simulink model "Controller"  (R2018b)
settings: configuration reference "control_config" (kept outside this file)
values from neighbouring files (symbols this model uses):
  CONTROL_EXPORT = Simulink.Parameter(CONTROL_EXPORT_VALUE)    [controller_model_init.m]
  CONTROL_PARAM = Simulink.Parameter(CONTROL_PARAM_VALUE)    [controller_model_init.m]
undefined symbols (not defined in the file or in its folder): actuator_cmd, CONTROL_CONST, ControlMode, DiscIntNeverNeededParam, timestamp, VehicleStatus
libraries: simulink x27, FMT_Model_Lib x7
(part 2 of 3)

== system Controller/Controller/Control_Allocation/Quadcopter_x/Roll_Pitch_Remix ==
  Effective_Matrix : Inport
  torque_cmd : Inport  Port=2
  throttle_cmd : Inport  Port=3
  Constant : Constant  Value=up_lim  OutDataTypeStr=single
  Constant1 : Constant  Value=lo_lim  OutDataTypeStr=single
  Max : MinMax  Function=max
  Max1 : MinMax
  Multiply : Product  Multiplication=Matrix(*)  OutDataTypeStr=single
  Multiply1 : Product  OutDataTypeStr=single
  PQ_Remix : Subsystem
  Reshape : Reshape  OutputDimensionality=Column vector (2-D)
  Saturation3 : Saturate  UpperLimit=1  LowerLimit=0
  Saturation4 : Saturate  UpperLimit=1  LowerLimit=0
  Selector : Selector  InputPortWidth=3  IndexOptions=Index vector (dialog)  Indices=[1 2]  OutputSizes=1
  Sum : Sum  Inputs=|++
  Sum1 : Sum  Inputs=|++
  Sum2 : Sum  Inputs=|++
  pq_column : Selector  NumberOfDimensions=2  InputPortWidth=3  IndexOptions=Select all,Index vector (dialog)  Indices=[1:4],[1 2]  OutputSizes=1,1
  pq_remix_throttle : Outport
  wires:
  Multiply1/1 -> Sum2/1
  Multiply/1 -> Multiply1/1, Sum/1
  Constant1/1 -> PQ_Remix/4(lo_min)
  Sum/1 -> Max/1, Max1/1  "pq_premix"
  Max1/1 -> PQ_Remix/2(min)
  pq_column/1 -> Multiply/1
  Constant/1 -> PQ_Remix/3(up_lim)
  throttle_cmd/1 -> PQ_Remix/5(force_z_cmd), Sum/2, Sum1/2
  Reshape/1 -> Multiply/2
  Sum2/1 -> Saturation4/1  "pq_remix"
  Sum1/1 -> Saturation3/1
  PQ_Remix/1(roll_pitch_scale) -> Multiply1/2  "roll_pitch_scale"
  Saturation3/1 -> Sum2/2
  Selector/1 -> Reshape/1
  Saturation4/1 -> pq_remix_throttle/1
  Max/1 -> PQ_Remix/1(max)
  PQ_Remix/2(floating_throttle) -> Sum1/1  "floating_throttle"
  Effective_Matrix/1 -> pq_column/1
  torque_cmd/1 -> Selector/1

== system Controller/Controller/Control_Allocation/Quadcopter_x/Yaw_Remix ==
  Effective_Matrix : Inport
  torque_cmd : Inport  Port=2
  pq_remix : Inport  Port=3
  Constant : Constant  Value=up_lim  OutDataTypeStr=single
  Constant1 : Constant  Value=lo_lim  OutDataTypeStr=single
  Multiply2 : Product  Multiplication=Matrix(*)  OutDataTypeStr=single
  R_Remix : MATLAB Function  TreatAsAtomicUnit=on
  Selector2 : Selector  InputPortWidth=3  IndexOptions=Index vector (dialog)  Indices=3  OutputSizes=1
  Sum3 : Sum  Inputs=|++
  Sum4 : Sum  Inputs=++|
  r_column : Selector  NumberOfDimensions=2  InputPortWidth=3  IndexOptions=Select all,Index vector (dialog)  Indices=[1:4],3  OutputSizes=1,1
  pqr_remix_throttle : Outport
  wires:
  Sum4/1 -> pqr_remix_throttle/1  "pqr_remix"
  Selector2/1 -> Multiply2/2
  Effective_Matrix/1 -> r_column/1
  torque_cmd/1 -> Selector2/1
  r_column/1 -> R_Remix/3(r_column), Multiply2/1
  Sum3/1 -> Sum4/2, R_Remix/4(motor_out)
  Multiply2/1 -> Sum3/1
  pq_remix/1 -> Sum3/2
  Constant/1 -> R_Remix/1(up_lim)
  Constant1/1 -> R_Remix/2(lo_lim)
  R_Remix/1(floating_yaw) -> Sum4/1  "floating_yaw"

== system Controller/Controller/Control_Allocation/Quadcopter_x/actuator_cmd_routing ==
  throttle_cmd : Inport
  status : Inport  Port=2
  Constant : Constant  Value=zeros(12,1)  VectorParams1D=off  OutDataTypeStr=uint16
  Constant2 : Constant  Value=1000  OutDataTypeStr=uint32
  Data Type Conversion : DataTypeConversion  OutDataTypeStr=uint16
  Disarm : Constant  Value=ones(4,1)*1000  VectorParams1D=off  OutDataTypeStr=uint16
  Gain3 : Gain  Gain=1000  OutDataTypeStr=uint32
  Multiport Switch : MultiPortSwitch  DataPortForDefault=Additional data port  DiagnosticForDefault=None
  Mux1 : Mux  Inputs=2
  Reshape : Reshape  OutputDimensionality=Customize  OutputDimensions=[16,1]
  Saturation5 : Saturate  UpperLimit=1  LowerLimit=0
  Standby : Constant  Value=ones(4,1)*1150  VectorParams1D=off  OutDataTypeStr=uint16
  Sum5 : Sum  Inputs=|++
  actuator_cmd : Outport
  wires:
  Disarm/1 -> Multiport Switch/5, Multiport Switch/2
  Reshape/1 -> actuator_cmd/1
  Constant/1 -> Mux1/2
  Standby/1 -> Multiport Switch/3
  Mux1/1 -> Reshape/1
  status/1 -> Multiport Switch/1
  Multiport Switch/1 -> Mux1/1
  Sum5/1 -> Data Type Conversion/1
  Saturation5/1 -> Gain3/1
  Gain3/1 -> Sum5/1
  Constant2/1 -> Sum5/2
  throttle_cmd/1 -> Saturation5/1
  Data Type Conversion/1 -> Multiport Switch/4

== system Controller/Controller/Horizontal_Control/Attitude_Controller/Inner_Loop ==
  euler_rate_cmd_radPs : Inport
  INS_Out : Inport  Port=2
  FMS_Out : Inport  Port=3
  Bus Selector : BusSelector  OutputSignals=reset
  Rate_Controller : Subsystem
  Signal_Convert : Subsystem
  Signal_Select : Subsystem
  rate_dot_cmd_B : Outport
  wires:
  euler_rate_cmd_radPs/1 -> Signal_Convert/2(euler_rate_cmd)
  Signal_Select/1(out) -> Rate_Controller/1(rate_cmd_radPs)
  Rate_Controller/1(rate_dot_cmd_B) -> rate_dot_cmd_B/1
  Bus Selector/1 -> Rate_Controller/3(reset)  "<reset>"
  INS_Out/1 -> Signal_Convert/3(INS_Out), Rate_Controller/2(INS_Out)
  FMS_Out/1 -> Signal_Convert/1(FMS_Out), Bus Selector/1, Signal_Select/1(FMS_Out)
  Signal_Convert/1(rate_cmd_radPs) -> Signal_Select/2(rate_cmd_radPs)

== system Controller/Controller/Horizontal_Control/Attitude_Controller/Outter_Loop ==
  att_cmd_rad : Inport
  INS_Out : Inport  Port=2
  FMS_Out : Inport  Port=3
  Attitude_Controller : Subsystem
  Signal_Select : Subsystem
  euler_rate_cmd_radPs : Outport
  wires:
  Signal_Select/1(out) -> Attitude_Controller/1(att_cmd_rad)
  FMS_Out/1 -> Signal_Select/2(FMS_Out)
  INS_Out/1 -> Attitude_Controller/2(INS_Out)
  Attitude_Controller/1(euler_rate_cmd_radPs) -> euler_rate_cmd_radPs/1
  att_cmd_rad/1 -> Signal_Select/1(att_cmd_rad)

== system Controller/Controller/Horizontal_Control/Velocity_Controller/Accel_to_Attitude_CMD ==
  note: Gain to resist
      | air drag
  accel_cmd_C_mPs2 : Inport
  Atan : Trigonometry  Operator=atan
  Divide : Product  Inputs=*/
  Gain1 : Gain  Gain=-1
  Mux : Mux  Inputs=2
  Mux1 : Mux  Inputs=2
  Mux2 : Mux  Inputs=2
  Saturation : Saturate  UpperLimit=CONTROL_PARAM.MC_ROLL_PITCH_LIM  LowerLimit=-CONTROL_PARAM.MC_ROLL_PITCH_LIM
  Selector : Selector  InputPortWidth=2  IndexOptions=Index vector (dialog)  Indices=1  OutputSizes=1
  Selector1 : Selector  InputPortWidth=2  IndexOptions=Index vector (dialog)  Indices=2  OutputSizes=1
  Vector Modulus : FMT_Model_Lib/Math/Vector Modulus
      settings: SourceProductName=FMT Toolbox
  g : Constant  Value=9.8055  OutDataTypeStr=single
  gain : Gain  Gain=1.1
  att_cmd_B_rad : Outport
  wires:
  Atan/1 -> Saturation/1
  g/1 -> Mux2/2, Mux1/1
  Divide/1 -> Atan/1
  Selector/1 -> Gain1/1
  gain/1 -> Selector1/1, Selector/1
  Gain1/1 -> Mux/2
  Saturation/1 -> att_cmd_B_rad/1
  Mux1/1 -> Divide/2
  Vector Modulus/1 -> Mux1/2
  Selector1/1 -> Mux2/1, Mux/1
  accel_cmd_C_mPs2/1 -> gain/1
  Mux/1 -> Divide/1
  Mux2/1 -> Vector Modulus/1

== system Controller/Controller/Horizontal_Control/Velocity_Controller/Error ==
  INS_Out : Inport
  FMS_Out : Inport  Port=2
  Bus Selector : BusSelector  OutputSignals=u_cmd,v_cmd
  Bus Selector1 : BusSelector  OutputSignals=flag
  Bus_Select : Subsystem
  Compare To Zero : simulink/Logic and Bit Operations/Compare To Zero  relop===  OutDataTypeStr=boolean
  Mux : Mux  Inputs=2
  Sum : Sum  Inputs=|+-
  Switch : Switch  Criteria=u2 > Threshold
  TD : Subsystem
  vel_valid : simulink/Logic and Bit Operations/Bitwise Operator  logicop=AND  UseBitMask=on  BitMask=bin2dec('10000')  BitMaskRealWorld=Stored Integer
  uv_err_C_mPs : Outport
  wires:
  FMS_Out/1 -> Bus Selector/1
  INS_Out/1 -> Bus Selector1/1, Bus_Select/1(INS_Out)
  Bus Selector/1 -> Mux/1  "<u_cmd>"
  Bus Selector/2 -> Mux/2  "<v_cmd>"
  Mux/1 -> Switch/1, TD/1(v)  "uv_cmd_C_mPs"
  Bus_Select/1(uv_est_C_mPs) -> Switch/3, Sum/2  "uv_est_C_mPs"
  Sum/1 -> uv_err_C_mPs/1  "uv_error_C_mPs"
  Bus Selector1/1 -> vel_valid/1  "<flag>"
  Switch/1 -> TD/2(v0)
  vel_valid/1 -> Compare To Zero/1
  Compare To Zero/1 -> Switch/2
  TD/1(v1) -> Sum/1  "uv_cmd_C_mPs"

== system Controller/Controller/Horizontal_Control/Velocity_Controller/PID_Controller ==
  uv_err_C_mPs : Inport
  reset : Inport  Port=2
  Add : Sum  Inputs=+++
  D_Control : Subsystem  mask{kd=CONTROL_PARAM.MC_VEL_XY_D, max_d=CONTROL_PARAM.MC_VEL_XY_D_MAX, min_d=CONTROL_PARAM.MC_VEL_XY_D_MIN}
  I_Control : Subsystem  mask{ki=CONTROL_PARAM.MC_VEL_XY_I, max_i=CONTROL_PARAM.MC_VEL_XY_I_MAX, min_i=CONTROL_PARAM.MC_VEL_XY_I_MIN}
  P_Control : Subsystem  mask{kp=CONTROL_PARAM.MC_VEL_XY_P}
  accel_cmd_C : Outport
  wires:
  uv_err_C_mPs/1 -> P_Control/1(err), I_Control/1(err), D_Control/1(err)
  reset/1 -> I_Control/2(reset), D_Control/2(reset)
  P_Control/1(p_out) -> Add/1  "accel_p_out"
  I_Control/1(i_out) -> Add/2  "accel_i_out"
  D_Control/1(d_out) -> Add/3  "accel_d_out"
  Add/1 -> accel_cmd_C/1

== system Controller/Controller/Horizontal_Control/Velocity_Controller/Signal_Select ==
  acc_cmd_in : Inport
  FMS_Out : Inport  Port=2
  Bus Selector : BusSelector  OutputSignals=ctrl_mode
  Offboard : simulink/Logic and Bit Operations/Compare To Constant  relop===  const=uint8(ControlMode.Offboard)  OutDataTypeStr=boolean
  Offboard_Signal_Select : Subsystem
  Switch : Switch  Criteria=u2 > Threshold
  acc_cmd_out : Outport
  wires:
  FMS_Out/1 -> Offboard_Signal_Select/1(FMS_Out), Bus Selector/1
  Bus Selector/1 -> Offboard/1  "<ctrl_mode>"
  Offboard/1 -> Switch/2
  Switch/1 -> acc_cmd_out/1
  acc_cmd_in/1 -> Offboard_Signal_Select/2(acc_cmd_in), Switch/3
  Offboard_Signal_Select/1(acc_cmd) -> Switch/1

== system Controller/Controller/Vertical_Control/Signal_Select/Offboard_Signal_Select ==
  FMS_Out : Inport
  throttle_cmd_in : Inport  Port=2
  Bias : Bias  Bias=-1
  Bus Selector1 : BusSelector  OutputSignals=cmd_mask
  Bus Selector2 : BusSelector  OutputSignals=throttle_cmd
  Gain : Gain  Gain=1/1000  OutDataTypeStr=single
  Switch : Switch  Criteria=u2 > Threshold
  cmd_throttle valid : simulink/Logic and Bit Operations/Bitwise Operator  logicop=AND  UseBitMask=on  BitMask=bin2dec('1000000000000')  BitMaskRealWorld=Stored Integer
  throttle_cmd_out : Outport
  wires:
  Switch/1 -> throttle_cmd_out/1
  cmd_throttle valid/1 -> Switch/2
  FMS_Out/1 -> Bus Selector2/1, Bus Selector1/1
  Bus Selector1/1 -> cmd_throttle valid/1  "<cmd_mask>"
  Bus Selector2/1 -> Gain/1  "<throttle_cmd>"
  throttle_cmd_in/1 -> Switch/3
  Gain/1 -> Bias/1
  Bias/1 -> Switch/1

== system Controller/Controller/Vertical_Control/Veloxity_Z_Controller/Boosted_Throttle ==
  thrust_cmd : Inport
  INS_Out : Inport  Port=2
  Bus Selector : BusSelector  OutputSignals=phi,theta
  Constant : Constant  OutDataTypeStr=single
  Cos : Trigonometry  Operator=cos
  Cos1 : Trigonometry  Operator=cos
  Divide : Product  Inputs=*/
  Gain : Gain  Gain=2
  Multiply : Product
  Multiply1 : Product  Inputs=3
  Saturation : Saturate  UpperLimit=1  LowerLimit=0
  Saturation1 : Saturate  UpperLimit=1  LowerLimit=0.5
  boosted_thrust : Outport
  wires:
  INS_Out/1 -> Bus Selector/1
  Bus Selector/1 -> Cos/1  "<phi>"
  Bus Selector/2 -> Cos1/1  "<theta>"
  Cos/1 -> Multiply/1
  Cos1/1 -> Multiply/2
  Multiply/1 -> Saturation1/1, Gain/1
  Gain/1 -> Saturation/1
  Saturation/1 -> Multiply1/3  "inverted_factor"
  Constant/1 -> Divide/1
  Divide/1 -> Multiply1/2  "boost_factor"
  Saturation1/1 -> Divide/2
  thrust_cmd/1 -> Multiply1/1
  Multiply1/1 -> boosted_thrust/1

== system Controller/Controller/Vertical_Control/Veloxity_Z_Controller/Error ==
  FMS_Out : Inport
  INS_Out : Inport  Port=2
  Bus Selector1 : BusSelector  OutputSignals=vd
  Bus Selector2 : BusSelector  OutputSignals=w_cmd
  Bus Selector3 : BusSelector  OutputSignals=flag
  Compare To Zero : simulink/Logic and Bit Operations/Compare To Zero  relop===  OutDataTypeStr=boolean
  Gain : Gain  Gain=-1  OutDataTypeStr=Inherit: Same as input
  Signal Copy1 : SignalConversion  OverrideOpt=off
  Sum1 : Sum  Inputs=|+-
  Switch : Switch  Criteria=u2 > Threshold
  TD : Subsystem
  vel_valid : simulink/Logic and Bit Operations/Bitwise Operator  logicop=AND  UseBitMask=on  BitMask=bin2dec('10000')  BitMaskRealWorld=Stored Integer
  az_cmd_C_mPs2 : Outport
  wires:
  Sum1/1 -> Gain/1  "w_error_C_mPs"
  FMS_Out/1 -> Bus Selector2/1
  TD/1(v1) -> Sum1/1  "w_cmd_C_mPs"
  Signal Copy1/1 -> Sum1/2  "w_est_C_mPs"
  Bus Selector2/1 -> Switch/1, TD/1(v)  "<w_cmd>"
  Gain/1 -> az_cmd_C_mPs2/1
  vel_valid/1 -> Compare To Zero/1
  Compare To Zero/1 -> Switch/2
  INS_Out/1 -> Bus Selector3/1, Bus Selector1/1
  Bus Selector3/1 -> vel_valid/1  "<flag>"
  Bus Selector1/1 -> Switch/3, Signal Copy1/1  "<vd>"
  Switch/1 -> TD/2(v0)

== system Controller/Controller/Vertical_Control/Veloxity_Z_Controller/PID_Controller ==
  az_cmd_C_mPs2 : Inport
  reset : Inport  Port=2
  prev_status : Inport  Port=3
  Add : Sum  Inputs=+++
  Compare To Constant : simulink/Logic and Bit Operations/Compare To Constant  relop=<  const=uint8(VehicleStatus.Arm)  OutDataTypeStr=boolean
  D_Control : Subsystem  mask{kd=CONTROL_PARAM.MC_VEL_Z_D, max_d=CONTROL_PARAM.MC_VEL_Z_D_MAX, min_d=CONTROL_PARAM.MC_VEL_Z_D_MIN}
  I_Control : Subsystem  mask{ki=CONTROL_PARAM.MC_VEL_Z_I, max_i=CONTROL_PARAM.MC_VEL_Z_I_MAX, min_i=CONTROL_PARAM.MC_VEL_Z_I_MIN}
  P_Control : Subsystem  mask{kp=CONTROL_PARAM.MC_VEL_Z_P}
  thrust_cmd : Outport
  wires:
  P_Control/1(p_out) -> Add/1  "thrust_p_out"
  I_Control/1(i_out) -> Add/2  "thrust_i_out"
  Add/1 -> thrust_cmd/1
  az_cmd_C_mPs2/1 -> D_Control/1(err), I_Control/1(err), P_Control/1(err)
  D_Control/1(d_out) -> Add/3  "thrust_d_out"
  Compare To Constant/1 -> I_Control/2(slow_start)
  reset/1 -> D_Control/2(reset), I_Control/3(reset)
  prev_status/1 -> Compare To Constant/1

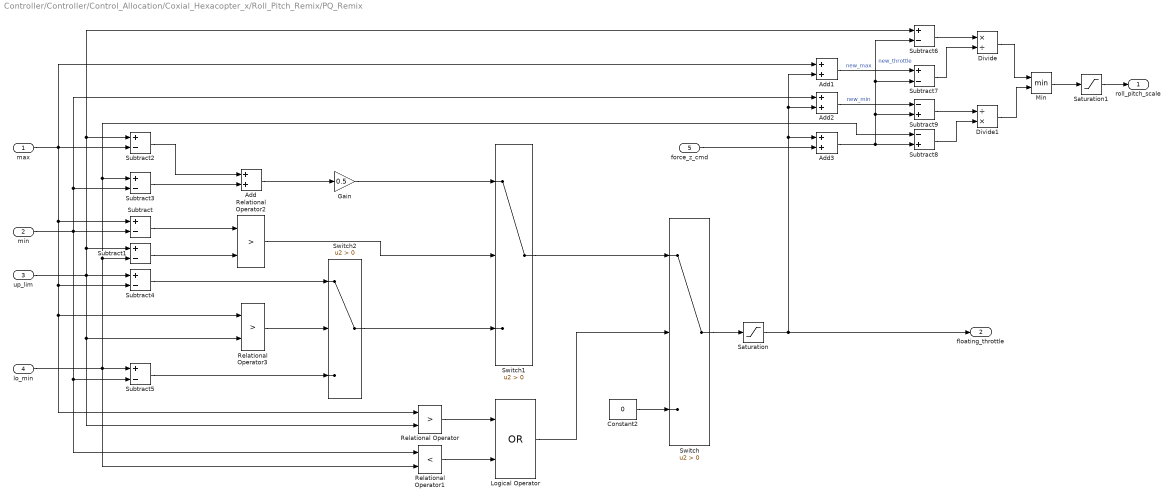
== system Controller/Controller/Control_Allocation/Coxial_Hexacopter_x/Roll_Pitch_Remix/PQ_Remix ==
  max : Inport
  min : Inport  Port=2
  up_lim : Inport  Port=3
  lo_min : Inport  Port=4
  force_z_cmd : Inport  Port=5
  Add{,1..3} (4 alike) : Sum
  Constant2 : Constant  Value=0  OutDataTypeStr=single
  Divide : Product  Inputs=*/
  Divide1 : Product  Inputs=/*
  Gain : Gain  Gain=0.5
  Logical Operator : Logic  Operator=OR  AllPortsSameDT=off  OutDataTypeStr=boolean
  Min : MinMax  Inputs=2
  Relational Operator : RelationalOperator  Operator=>  OutDataTypeStr=boolean  RndMeth=Simplest
  Relational Operator1 : RelationalOperator  Operator=<  OutDataTypeStr=boolean  RndMeth=Simplest
  Relational Operator2 : RelationalOperator  Operator=>  OutDataTypeStr=boolean  RndMeth=Simplest
  Relational Operator3 : RelationalOperator  Operator=>  OutDataTypeStr=boolean  RndMeth=Simplest
  Saturation : Saturate  UpperLimit=0.2  LowerLimit=-0.2
  Saturation1 : Saturate  UpperLimit=1  LowerLimit=0.5
  Subtract{,1..7} (8 alike) : Sum  Inputs=+-
  Subtract8 : Sum  Inputs=-+
  Subtract9 : Sum  Inputs=-+
  Switch : Switch  Criteria=u2 > Threshold
  Switch1 : Switch  Criteria=u2 > Threshold
  Switch2 : Switch  Criteria=u2 > Threshold
  roll_pitch_scale : Outport
  floating_throttle : Outport  Port=2
  wires:
  max/1 -> Subtract/1, Relational Operator3/1, Relational Operator/1, Subtract4/2, Add1/1, Subtract2/2
  up_lim/1 -> Relational Operator/2, Relational Operator3/2, Subtract6/1, Subtract2/1, Subtract1/1, Subtract4/1
  min/1 -> Add2/1, Subtract3/2, Subtract/2, Relational Operator1/1, Subtract5/2
  lo_min/1 -> Subtract8/1, Subtract3/1, Subtract1/2, Relational Operator1/2, Subtract5/1
  Relational Operator/1 -> Logical Operator/1
  Relational Operator1/1 -> Logical Operator/2
  Logical Operator/1 -> Switch/2
  Constant2/1 -> Switch/3
  Subtract/1 -> Relational Operator2/1
  Subtract1/1 -> Relational Operator2/2
  Relational Operator2/1 -> Switch1/2
  Subtract2/1 -> Add/1
  Subtract3/1 -> Add/2
  Add/1 -> Gain/1
  Gain/1 -> Switch1/1
  Relational Operator3/1 -> Switch2/2
  Subtract4/1 -> Switch2/1
  Switch1/1 -> Switch/1
  Switch2/1 -> Switch1/3
  Subtract5/1 -> Switch2/3
  Switch/1 -> Saturation/1
  force_z_cmd/1 -> Add3/2
  Add1/1 -> Subtract7/1  "new_max"
  Add2/1 -> Subtract9/1  "new_min"
  Add3/1 -> Subtract7/2, Subtract6/2, Subtract9/2, Subtract8/2  "new_throttle"
  Subtract6/1 -> Divide/1
  Subtract7/1 -> Divide/2
  Subtract8/1 -> Divide1/2
  Subtract9/1 -> Divide1/1
  Divide/1 -> Min/1
  Divide1/1 -> Min/2
  Min/1 -> Saturation1/1
  Saturation1/1 -> roll_pitch_scale/1
  Saturation/1 -> Add3/1, Add2/2, Add1/2, floating_throttle/1

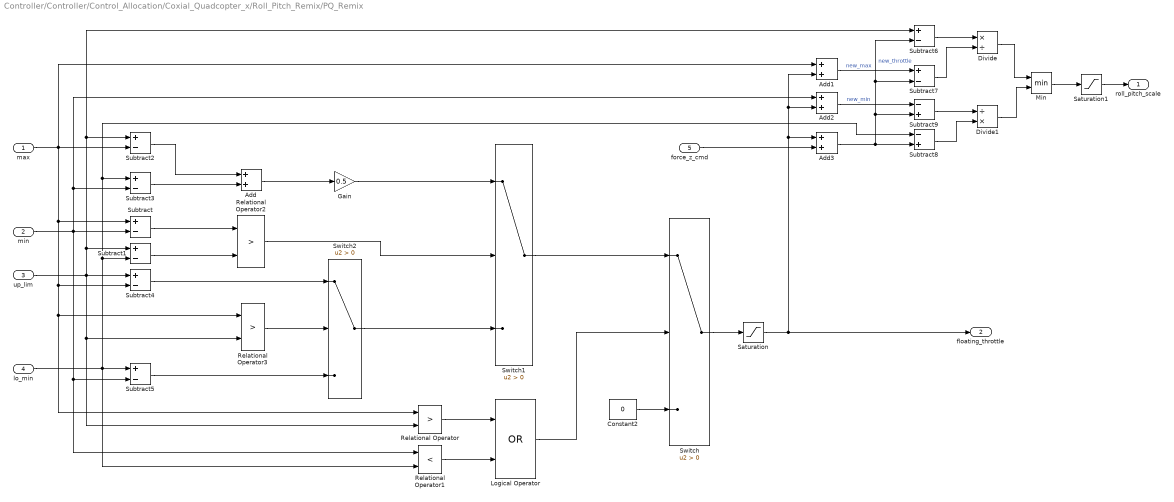
== system Controller/Controller/Control_Allocation/Coxial_Quadcopter_x/Roll_Pitch_Remix/PQ_Remix ==
  max : Inport
  min : Inport  Port=2
  up_lim : Inport  Port=3
  lo_min : Inport  Port=4
  force_z_cmd : Inport  Port=5
  Add{,1..3} (4 alike) : Sum
  Constant2 : Constant  Value=0  OutDataTypeStr=single
  Divide : Product  Inputs=*/
  Divide1 : Product  Inputs=/*
  Gain : Gain  Gain=0.5
  Logical Operator : Logic  Operator=OR  AllPortsSameDT=off  OutDataTypeStr=boolean
  Min : MinMax  Inputs=2
  Relational Operator : RelationalOperator  Operator=>  OutDataTypeStr=boolean  RndMeth=Simplest
  Relational Operator1 : RelationalOperator  Operator=<  OutDataTypeStr=boolean  RndMeth=Simplest
  Relational Operator2 : RelationalOperator  Operator=>  OutDataTypeStr=boolean  RndMeth=Simplest
  Relational Operator3 : RelationalOperator  Operator=>  OutDataTypeStr=boolean  RndMeth=Simplest
  Saturation : Saturate  UpperLimit=0.2  LowerLimit=-0.2
  Saturation1 : Saturate  UpperLimit=1  LowerLimit=0.5
  Subtract{,1..7} (8 alike) : Sum  Inputs=+-
  Subtract8 : Sum  Inputs=-+
  Subtract9 : Sum  Inputs=-+
  Switch : Switch  Criteria=u2 > Threshold
  Switch1 : Switch  Criteria=u2 > Threshold
  Switch2 : Switch  Criteria=u2 > Threshold
  roll_pitch_scale : Outport
  floating_throttle : Outport  Port=2
  wires:
  max/1 -> Subtract/1, Relational Operator3/1, Relational Operator/1, Subtract4/2, Add1/1, Subtract2/2
  up_lim/1 -> Relational Operator/2, Relational Operator3/2, Subtract6/1, Subtract2/1, Subtract1/1, Subtract4/1
  min/1 -> Add2/1, Subtract3/2, Subtract/2, Relational Operator1/1, Subtract5/2
  lo_min/1 -> Subtract8/1, Subtract3/1, Subtract1/2, Relational Operator1/2, Subtract5/1
  Relational Operator/1 -> Logical Operator/1
  Relational Operator1/1 -> Logical Operator/2
  Logical Operator/1 -> Switch/2
  Constant2/1 -> Switch/3
  Subtract/1 -> Relational Operator2/1
  Subtract1/1 -> Relational Operator2/2
  Relational Operator2/1 -> Switch1/2
  Subtract2/1 -> Add/1
  Subtract3/1 -> Add/2
  Add/1 -> Gain/1
  Gain/1 -> Switch1/1
  Relational Operator3/1 -> Switch2/2
  Subtract4/1 -> Switch2/1
  Switch1/1 -> Switch/1
  Switch2/1 -> Switch1/3
  Subtract5/1 -> Switch2/3
  Switch/1 -> Saturation/1
  force_z_cmd/1 -> Add3/2
  Add1/1 -> Subtract7/1  "new_max"
  Add2/1 -> Subtract9/1  "new_min"
  Add3/1 -> Subtract7/2, Subtract6/2, Subtract9/2, Subtract8/2  "new_throttle"
  Subtract6/1 -> Divide/1
  Subtract7/1 -> Divide/2
  Subtract8/1 -> Divide1/2
  Subtract9/1 -> Divide1/1
  Divide/1 -> Min/1
  Divide1/1 -> Min/2
  Min/1 -> Saturation1/1
  Saturation1/1 -> roll_pitch_scale/1
  Saturation/1 -> Add3/1, Add2/2, Add1/2, floating_throttle/1

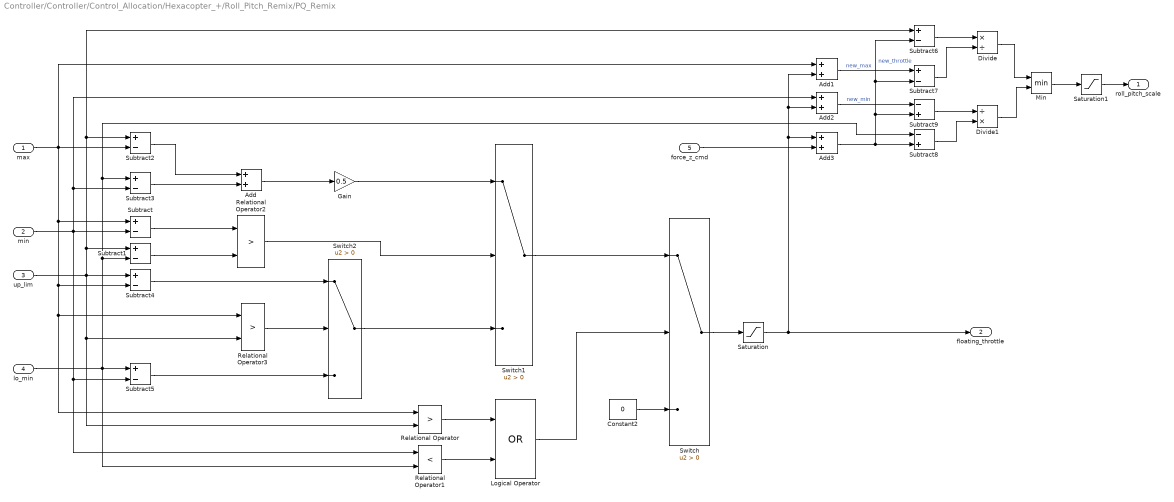
== system Controller/Controller/Control_Allocation/Hexacopter_+/Roll_Pitch_Remix/PQ_Remix ==
  max : Inport
  min : Inport  Port=2
  up_lim : Inport  Port=3
  lo_min : Inport  Port=4
  force_z_cmd : Inport  Port=5
  Add{,1..3} (4 alike) : Sum
  Constant2 : Constant  Value=0  OutDataTypeStr=single
  Divide : Product  Inputs=*/
  Divide1 : Product  Inputs=/*
  Gain : Gain  Gain=0.5
  Logical Operator : Logic  Operator=OR  AllPortsSameDT=off  OutDataTypeStr=boolean
  Min : MinMax  Inputs=2
  Relational Operator : RelationalOperator  Operator=>  OutDataTypeStr=boolean  RndMeth=Simplest
  Relational Operator1 : RelationalOperator  Operator=<  OutDataTypeStr=boolean  RndMeth=Simplest
  Relational Operator2 : RelationalOperator  Operator=>  OutDataTypeStr=boolean  RndMeth=Simplest
  Relational Operator3 : RelationalOperator  Operator=>  OutDataTypeStr=boolean  RndMeth=Simplest
  Saturation : Saturate  UpperLimit=0.2  LowerLimit=-0.2
  Saturation1 : Saturate  UpperLimit=1  LowerLimit=0.5
  Subtract{,1..7} (8 alike) : Sum  Inputs=+-
  Subtract8 : Sum  Inputs=-+
  Subtract9 : Sum  Inputs=-+
  Switch : Switch  Criteria=u2 > Threshold
  Switch1 : Switch  Criteria=u2 > Threshold
  Switch2 : Switch  Criteria=u2 > Threshold
  roll_pitch_scale : Outport
  floating_throttle : Outport  Port=2
  wires:
  max/1 -> Subtract/1, Relational Operator3/1, Relational Operator/1, Subtract4/2, Add1/1, Subtract2/2
  up_lim/1 -> Relational Operator/2, Relational Operator3/2, Subtract6/1, Subtract2/1, Subtract1/1, Subtract4/1
  min/1 -> Add2/1, Subtract3/2, Subtract/2, Relational Operator1/1, Subtract5/2
  lo_min/1 -> Subtract8/1, Subtract3/1, Subtract1/2, Relational Operator1/2, Subtract5/1
  Relational Operator/1 -> Logical Operator/1
  Relational Operator1/1 -> Logical Operator/2
  Logical Operator/1 -> Switch/2
  Constant2/1 -> Switch/3
  Subtract/1 -> Relational Operator2/1
  Subtract1/1 -> Relational Operator2/2
  Relational Operator2/1 -> Switch1/2
  Subtract2/1 -> Add/1
  Subtract3/1 -> Add/2
  Add/1 -> Gain/1
  Gain/1 -> Switch1/1
  Relational Operator3/1 -> Switch2/2
  Subtract4/1 -> Switch2/1
  Switch1/1 -> Switch/1
  Switch2/1 -> Switch1/3
  Subtract5/1 -> Switch2/3
  Switch/1 -> Saturation/1
  force_z_cmd/1 -> Add3/2
  Add1/1 -> Subtract7/1  "new_max"
  Add2/1 -> Subtract9/1  "new_min"
  Add3/1 -> Subtract7/2, Subtract6/2, Subtract9/2, Subtract8/2  "new_throttle"
  Subtract6/1 -> Divide/1
  Subtract7/1 -> Divide/2
  Subtract8/1 -> Divide1/2
  Subtract9/1 -> Divide1/1
  Divide/1 -> Min/1
  Divide1/1 -> Min/2
  Min/1 -> Saturation1/1
  Saturation1/1 -> roll_pitch_scale/1
  Saturation/1 -> Add3/1, Add2/2, Add1/2, floating_throttle/1

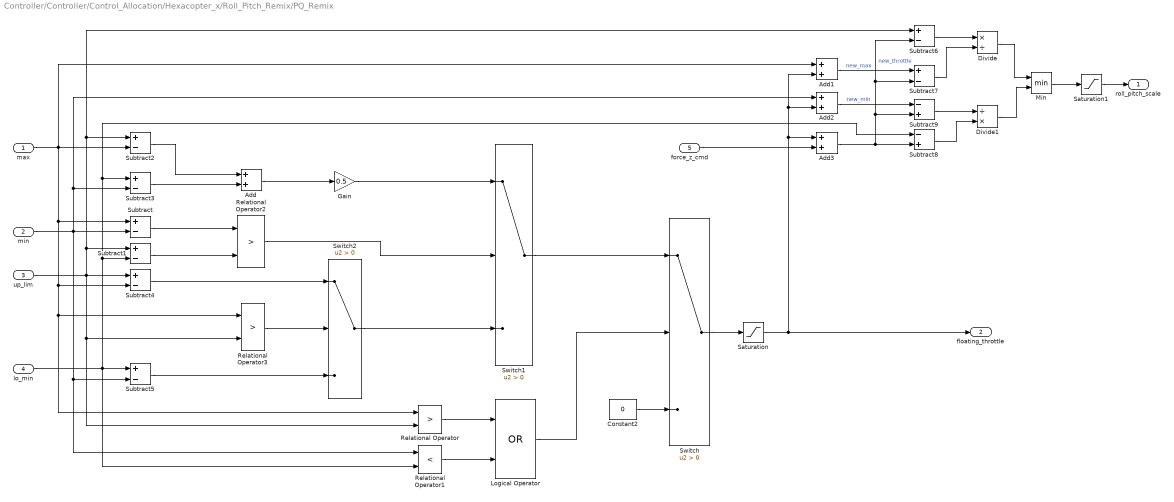
== system Controller/Controller/Control_Allocation/Hexacopter_x/Roll_Pitch_Remix/PQ_Remix ==
  max : Inport
  min : Inport  Port=2
  up_lim : Inport  Port=3
  lo_min : Inport  Port=4
  force_z_cmd : Inport  Port=5
  Add{,1..3} (4 alike) : Sum
  Constant2 : Constant  Value=0  OutDataTypeStr=single
  Divide : Product  Inputs=*/
  Divide1 : Product  Inputs=/*
  Gain : Gain  Gain=0.5
  Logical Operator : Logic  Operator=OR  AllPortsSameDT=off  OutDataTypeStr=boolean
  Min : MinMax  Inputs=2
  Relational Operator : RelationalOperator  Operator=>  OutDataTypeStr=boolean  RndMeth=Simplest
  Relational Operator1 : RelationalOperator  Operator=<  OutDataTypeStr=boolean  RndMeth=Simplest
  Relational Operator2 : RelationalOperator  Operator=>  OutDataTypeStr=boolean  RndMeth=Simplest
  Relational Operator3 : RelationalOperator  Operator=>  OutDataTypeStr=boolean  RndMeth=Simplest
  Saturation : Saturate  UpperLimit=0.2  LowerLimit=-0.2
  Saturation1 : Saturate  UpperLimit=1  LowerLimit=0.5
  Subtract{,1..7} (8 alike) : Sum  Inputs=+-
  Subtract8 : Sum  Inputs=-+
  Subtract9 : Sum  Inputs=-+
  Switch : Switch  Criteria=u2 > Threshold
  Switch1 : Switch  Criteria=u2 > Threshold
  Switch2 : Switch  Criteria=u2 > Threshold
  roll_pitch_scale : Outport
  floating_throttle : Outport  Port=2
  wires:
  max/1 -> Subtract/1, Relational Operator3/1, Relational Operator/1, Subtract4/2, Add1/1, Subtract2/2
  up_lim/1 -> Relational Operator/2, Relational Operator3/2, Subtract6/1, Subtract2/1, Subtract1/1, Subtract4/1
  min/1 -> Add2/1, Subtract3/2, Subtract/2, Relational Operator1/1, Subtract5/2
  lo_min/1 -> Subtract8/1, Subtract3/1, Subtract1/2, Relational Operator1/2, Subtract5/1
  Relational Operator/1 -> Logical Operator/1
  Relational Operator1/1 -> Logical Operator/2
  Logical Operator/1 -> Switch/2
  Constant2/1 -> Switch/3
  Subtract/1 -> Relational Operator2/1
  Subtract1/1 -> Relational Operator2/2
  Relational Operator2/1 -> Switch1/2
  Subtract2/1 -> Add/1
  Subtract3/1 -> Add/2
  Add/1 -> Gain/1
  Gain/1 -> Switch1/1
  Relational Operator3/1 -> Switch2/2
  Subtract4/1 -> Switch2/1
  Switch1/1 -> Switch/1
  Switch2/1 -> Switch1/3
  Subtract5/1 -> Switch2/3
  Switch/1 -> Saturation/1
  force_z_cmd/1 -> Add3/2
  Add1/1 -> Subtract7/1  "new_max"
  Add2/1 -> Subtract9/1  "new_min"
  Add3/1 -> Subtract7/2, Subtract6/2, Subtract9/2, Subtract8/2  "new_throttle"
  Subtract6/1 -> Divide/1
  Subtract7/1 -> Divide/2
  Subtract8/1 -> Divide1/2
  Subtract9/1 -> Divide1/1
  Divide/1 -> Min/1
  Divide1/1 -> Min/2
  Min/1 -> Saturation1/1
  Saturation1/1 -> roll_pitch_scale/1
  Saturation/1 -> Add3/1, Add2/2, Add1/2, floating_throttle/1

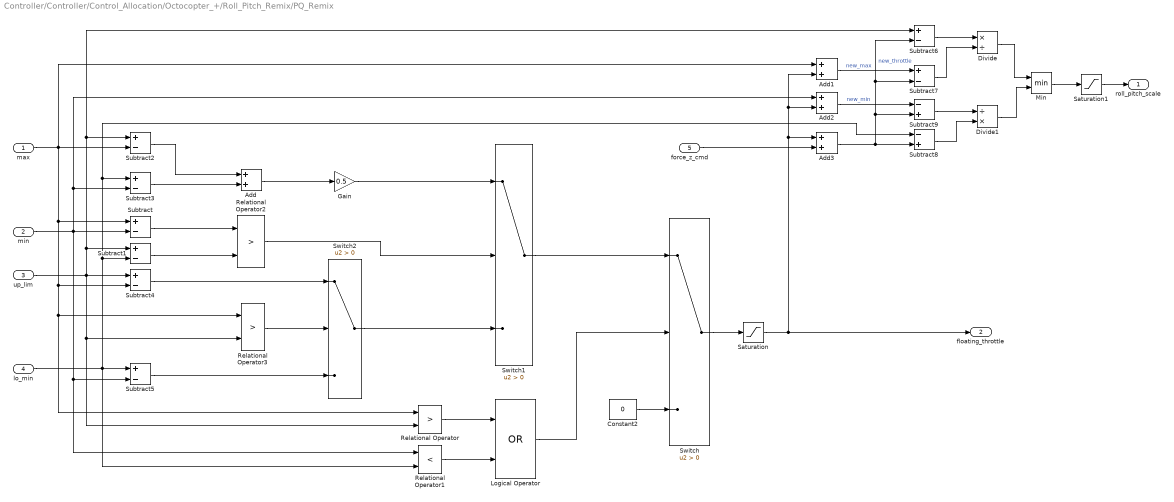
== system Controller/Controller/Control_Allocation/Octocopter_+/Roll_Pitch_Remix/PQ_Remix ==
  max : Inport
  min : Inport  Port=2
  up_lim : Inport  Port=3
  lo_min : Inport  Port=4
  force_z_cmd : Inport  Port=5
  Add{,1..3} (4 alike) : Sum
  Constant2 : Constant  Value=0  OutDataTypeStr=single
  Divide : Product  Inputs=*/
  Divide1 : Product  Inputs=/*
  Gain : Gain  Gain=0.5
  Logical Operator : Logic  Operator=OR  AllPortsSameDT=off  OutDataTypeStr=boolean
  Min : MinMax  Inputs=2
  Relational Operator : RelationalOperator  Operator=>  OutDataTypeStr=boolean  RndMeth=Simplest
  Relational Operator1 : RelationalOperator  Operator=<  OutDataTypeStr=boolean  RndMeth=Simplest
  Relational Operator2 : RelationalOperator  Operator=>  OutDataTypeStr=boolean  RndMeth=Simplest
  Relational Operator3 : RelationalOperator  Operator=>  OutDataTypeStr=boolean  RndMeth=Simplest
  Saturation : Saturate  UpperLimit=0.2  LowerLimit=-0.2
  Saturation1 : Saturate  UpperLimit=1  LowerLimit=0.5
  Subtract{,1..7} (8 alike) : Sum  Inputs=+-
  Subtract8 : Sum  Inputs=-+
  Subtract9 : Sum  Inputs=-+
  Switch : Switch  Criteria=u2 > Threshold
  Switch1 : Switch  Criteria=u2 > Threshold
  Switch2 : Switch  Criteria=u2 > Threshold
  roll_pitch_scale : Outport
  floating_throttle : Outport  Port=2
  wires:
  max/1 -> Subtract/1, Relational Operator3/1, Relational Operator/1, Subtract4/2, Add1/1, Subtract2/2
  up_lim/1 -> Relational Operator/2, Relational Operator3/2, Subtract6/1, Subtract2/1, Subtract1/1, Subtract4/1
  min/1 -> Add2/1, Subtract3/2, Subtract/2, Relational Operator1/1, Subtract5/2
  lo_min/1 -> Subtract8/1, Subtract3/1, Subtract1/2, Relational Operator1/2, Subtract5/1
  Relational Operator/1 -> Logical Operator/1
  Relational Operator1/1 -> Logical Operator/2
  Logical Operator/1 -> Switch/2
  Constant2/1 -> Switch/3
  Subtract/1 -> Relational Operator2/1
  Subtract1/1 -> Relational Operator2/2
  Relational Operator2/1 -> Switch1/2
  Subtract2/1 -> Add/1
  Subtract3/1 -> Add/2
  Add/1 -> Gain/1
  Gain/1 -> Switch1/1
  Relational Operator3/1 -> Switch2/2
  Subtract4/1 -> Switch2/1
  Switch1/1 -> Switch/1
  Switch2/1 -> Switch1/3
  Subtract5/1 -> Switch2/3
  Switch/1 -> Saturation/1
  force_z_cmd/1 -> Add3/2
  Add1/1 -> Subtract7/1  "new_max"
  Add2/1 -> Subtract9/1  "new_min"
  Add3/1 -> Subtract7/2, Subtract6/2, Subtract9/2, Subtract8/2  "new_throttle"
  Subtract6/1 -> Divide/1
  Subtract7/1 -> Divide/2
  Subtract8/1 -> Divide1/2
  Subtract9/1 -> Divide1/1
  Divide/1 -> Min/1
  Divide1/1 -> Min/2
  Min/1 -> Saturation1/1
  Saturation1/1 -> roll_pitch_scale/1
  Saturation/1 -> Add3/1, Add2/2, Add1/2, floating_throttle/1

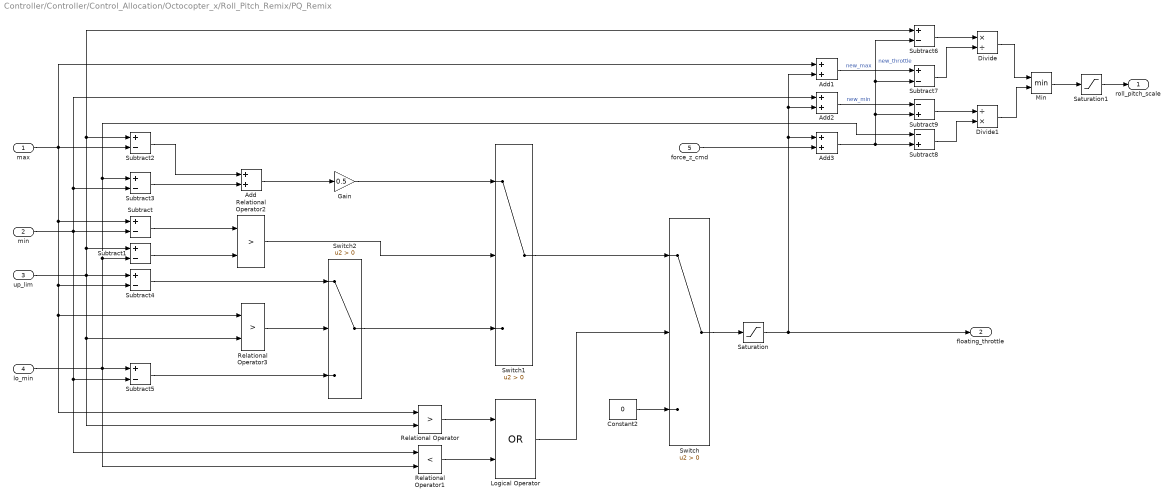
== system Controller/Controller/Control_Allocation/Octocopter_x/Roll_Pitch_Remix/PQ_Remix ==
  max : Inport
  min : Inport  Port=2
  up_lim : Inport  Port=3
  lo_min : Inport  Port=4
  force_z_cmd : Inport  Port=5
  Add{,1..3} (4 alike) : Sum
  Constant2 : Constant  Value=0  OutDataTypeStr=single
  Divide : Product  Inputs=*/
  Divide1 : Product  Inputs=/*
  Gain : Gain  Gain=0.5
  Logical Operator : Logic  Operator=OR  AllPortsSameDT=off  OutDataTypeStr=boolean
  Min : MinMax  Inputs=2
  Relational Operator : RelationalOperator  Operator=>  OutDataTypeStr=boolean  RndMeth=Simplest
  Relational Operator1 : RelationalOperator  Operator=<  OutDataTypeStr=boolean  RndMeth=Simplest
  Relational Operator2 : RelationalOperator  Operator=>  OutDataTypeStr=boolean  RndMeth=Simplest
  Relational Operator3 : RelationalOperator  Operator=>  OutDataTypeStr=boolean  RndMeth=Simplest
  Saturation : Saturate  UpperLimit=0.2  LowerLimit=-0.2
  Saturation1 : Saturate  UpperLimit=1  LowerLimit=0.5
  Subtract{,1..7} (8 alike) : Sum  Inputs=+-
  Subtract8 : Sum  Inputs=-+
  Subtract9 : Sum  Inputs=-+
  Switch : Switch  Criteria=u2 > Threshold
  Switch1 : Switch  Criteria=u2 > Threshold
  Switch2 : Switch  Criteria=u2 > Threshold
  roll_pitch_scale : Outport
  floating_throttle : Outport  Port=2
  wires:
  max/1 -> Subtract/1, Relational Operator3/1, Relational Operator/1, Subtract4/2, Add1/1, Subtract2/2
  up_lim/1 -> Relational Operator/2, Relational Operator3/2, Subtract6/1, Subtract2/1, Subtract1/1, Subtract4/1
  min/1 -> Add2/1, Subtract3/2, Subtract/2, Relational Operator1/1, Subtract5/2
  lo_min/1 -> Subtract8/1, Subtract3/1, Subtract1/2, Relational Operator1/2, Subtract5/1
  Relational Operator/1 -> Logical Operator/1
  Relational Operator1/1 -> Logical Operator/2
  Logical Operator/1 -> Switch/2
  Constant2/1 -> Switch/3
  Subtract/1 -> Relational Operator2/1
  Subtract1/1 -> Relational Operator2/2
  Relational Operator2/1 -> Switch1/2
  Subtract2/1 -> Add/1
  Subtract3/1 -> Add/2
  Add/1 -> Gain/1
  Gain/1 -> Switch1/1
  Relational Operator3/1 -> Switch2/2
  Subtract4/1 -> Switch2/1
  Switch1/1 -> Switch/1
  Switch2/1 -> Switch1/3
  Subtract5/1 -> Switch2/3
  Switch/1 -> Saturation/1
  force_z_cmd/1 -> Add3/2
  Add1/1 -> Subtract7/1  "new_max"
  Add2/1 -> Subtract9/1  "new_min"
  Add3/1 -> Subtract7/2, Subtract6/2, Subtract9/2, Subtract8/2  "new_throttle"
  Subtract6/1 -> Divide/1
  Subtract7/1 -> Divide/2
  Subtract8/1 -> Divide1/2
  Subtract9/1 -> Divide1/1
  Divide/1 -> Min/1
  Divide1/1 -> Min/2
  Min/1 -> Saturation1/1
  Saturation1/1 -> roll_pitch_scale/1
  Saturation/1 -> Add3/1, Add2/2, Add1/2, floating_throttle/1

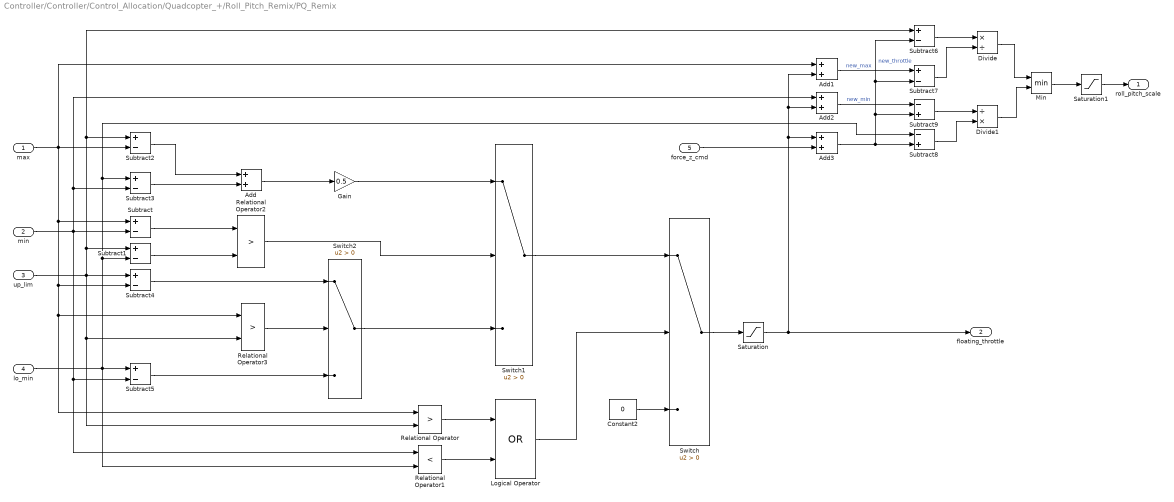
== system Controller/Controller/Control_Allocation/Quadcopter_+/Roll_Pitch_Remix/PQ_Remix ==
  max : Inport
  min : Inport  Port=2
  up_lim : Inport  Port=3
  lo_min : Inport  Port=4
  force_z_cmd : Inport  Port=5
  Add{,1..3} (4 alike) : Sum
  Constant2 : Constant  Value=0  OutDataTypeStr=single
  Divide : Product  Inputs=*/
  Divide1 : Product  Inputs=/*
  Gain : Gain  Gain=0.5
  Logical Operator : Logic  Operator=OR  AllPortsSameDT=off  OutDataTypeStr=boolean
  Min : MinMax  Inputs=2
  Relational Operator : RelationalOperator  Operator=>  OutDataTypeStr=boolean  RndMeth=Simplest
  Relational Operator1 : RelationalOperator  Operator=<  OutDataTypeStr=boolean  RndMeth=Simplest
  Relational Operator2 : RelationalOperator  Operator=>  OutDataTypeStr=boolean  RndMeth=Simplest
  Relational Operator3 : RelationalOperator  Operator=>  OutDataTypeStr=boolean  RndMeth=Simplest
  Saturation : Saturate  UpperLimit=0.2  LowerLimit=-0.2
  Saturation1 : Saturate  UpperLimit=1  LowerLimit=0.5
  Subtract{,1..7} (8 alike) : Sum  Inputs=+-
  Subtract8 : Sum  Inputs=-+
  Subtract9 : Sum  Inputs=-+
  Switch : Switch  Criteria=u2 > Threshold
  Switch1 : Switch  Criteria=u2 > Threshold
  Switch2 : Switch  Criteria=u2 > Threshold
  roll_pitch_scale : Outport
  floating_throttle : Outport  Port=2
  wires:
  max/1 -> Subtract/1, Relational Operator3/1, Relational Operator/1, Subtract4/2, Add1/1, Subtract2/2
  up_lim/1 -> Relational Operator/2, Relational Operator3/2, Subtract6/1, Subtract2/1, Subtract1/1, Subtract4/1
  min/1 -> Add2/1, Subtract3/2, Subtract/2, Relational Operator1/1, Subtract5/2
  lo_min/1 -> Subtract8/1, Subtract3/1, Subtract1/2, Relational Operator1/2, Subtract5/1
  Relational Operator/1 -> Logical Operator/1
  Relational Operator1/1 -> Logical Operator/2
  Logical Operator/1 -> Switch/2
  Constant2/1 -> Switch/3
  Subtract/1 -> Relational Operator2/1
  Subtract1/1 -> Relational Operator2/2
  Relational Operator2/1 -> Switch1/2
  Subtract2/1 -> Add/1
  Subtract3/1 -> Add/2
  Add/1 -> Gain/1
  Gain/1 -> Switch1/1
  Relational Operator3/1 -> Switch2/2
  Subtract4/1 -> Switch2/1
  Switch1/1 -> Switch/1
  Switch2/1 -> Switch1/3
  Subtract5/1 -> Switch2/3
  Switch/1 -> Saturation/1
  force_z_cmd/1 -> Add3/2
  Add1/1 -> Subtract7/1  "new_max"
  Add2/1 -> Subtract9/1  "new_min"
  Add3/1 -> Subtract7/2, Subtract6/2, Subtract9/2, Subtract8/2  "new_throttle"
  Subtract6/1 -> Divide/1
  Subtract7/1 -> Divide/2
  Subtract8/1 -> Divide1/2
  Subtract9/1 -> Divide1/1
  Divide/1 -> Min/1
  Divide1/1 -> Min/2
  Min/1 -> Saturation1/1
  Saturation1/1 -> roll_pitch_scale/1
  Saturation/1 -> Add3/1, Add2/2, Add1/2, floating_throttle/1

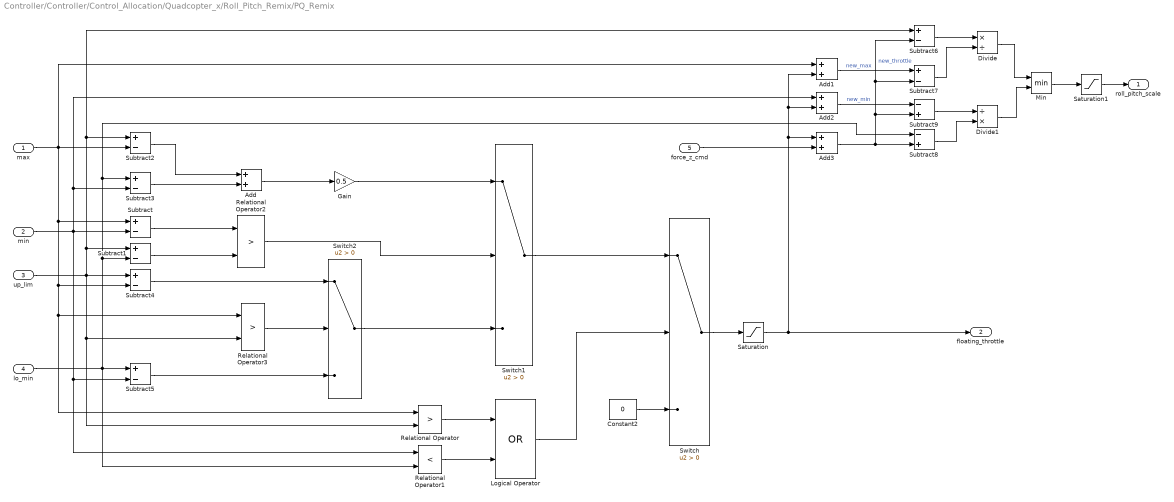
== system Controller/Controller/Control_Allocation/Quadcopter_x/Roll_Pitch_Remix/PQ_Remix ==
  max : Inport
  min : Inport  Port=2
  up_lim : Inport  Port=3
  lo_min : Inport  Port=4
  force_z_cmd : Inport  Port=5
  Add{,1..3} (4 alike) : Sum
  Constant2 : Constant  Value=0  OutDataTypeStr=single
  Divide : Product  Inputs=*/
  Divide1 : Product  Inputs=/*
  Gain : Gain  Gain=0.5
  Logical Operator : Logic  Operator=OR  AllPortsSameDT=off  OutDataTypeStr=boolean
  Min : MinMax  Inputs=2
  Relational Operator : RelationalOperator  Operator=>  OutDataTypeStr=boolean  RndMeth=Simplest
  Relational Operator1 : RelationalOperator  Operator=<  OutDataTypeStr=boolean  RndMeth=Simplest
  Relational Operator2 : RelationalOperator  Operator=>  OutDataTypeStr=boolean  RndMeth=Simplest
  Relational Operator3 : RelationalOperator  Operator=>  OutDataTypeStr=boolean  RndMeth=Simplest
  Saturation : Saturate  UpperLimit=0.2  LowerLimit=-0.2
  Saturation1 : Saturate  UpperLimit=1  LowerLimit=0.5
  Subtract{,1..7} (8 alike) : Sum  Inputs=+-
  Subtract8 : Sum  Inputs=-+
  Subtract9 : Sum  Inputs=-+
  Switch : Switch  Criteria=u2 > Threshold
  Switch1 : Switch  Criteria=u2 > Threshold
  Switch2 : Switch  Criteria=u2 > Threshold
  roll_pitch_scale : Outport
  floating_throttle : Outport  Port=2
  wires:
  max/1 -> Subtract/1, Relational Operator3/1, Relational Operator/1, Subtract4/2, Add1/1, Subtract2/2
  up_lim/1 -> Relational Operator/2, Relational Operator3/2, Subtract6/1, Subtract2/1, Subtract1/1, Subtract4/1
  min/1 -> Add2/1, Subtract3/2, Subtract/2, Relational Operator1/1, Subtract5/2
  lo_min/1 -> Subtract8/1, Subtract3/1, Subtract1/2, Relational Operator1/2, Subtract5/1
  Relational Operator/1 -> Logical Operator/1
  Relational Operator1/1 -> Logical Operator/2
  Logical Operator/1 -> Switch/2
  Constant2/1 -> Switch/3
  Subtract/1 -> Relational Operator2/1
  Subtract1/1 -> Relational Operator2/2
  Relational Operator2/1 -> Switch1/2
  Subtract2/1 -> Add/1
  Subtract3/1 -> Add/2
  Add/1 -> Gain/1
  Gain/1 -> Switch1/1
  Relational Operator3/1 -> Switch2/2
  Subtract4/1 -> Switch2/1
  Switch1/1 -> Switch/1
  Switch2/1 -> Switch1/3
  Subtract5/1 -> Switch2/3
  Switch/1 -> Saturation/1
  force_z_cmd/1 -> Add3/2
  Add1/1 -> Subtract7/1  "new_max"
  Add2/1 -> Subtract9/1  "new_min"
  Add3/1 -> Subtract7/2, Subtract6/2, Subtract9/2, Subtract8/2  "new_throttle"
  Subtract6/1 -> Divide/1
  Subtract7/1 -> Divide/2
  Subtract8/1 -> Divide1/2
  Subtract9/1 -> Divide1/1
  Divide/1 -> Min/1
  Divide1/1 -> Min/2
  Min/1 -> Saturation1/1
  Saturation1/1 -> roll_pitch_scale/1
  Saturation/1 -> Add3/1, Add2/2, Add1/2, floating_throttle/1

== system Controller/Controller/Horizontal_Control/Attitude_Controller/Inner_Loop/Rate_Controller ==
  rate_cmd_radPs : Inport
  INS_Out : Inport  Port=2
  reset : Inport  Port=3
  Error : Subsystem
  Feedforward_Controller : Subsystem
  PID_Controller : Subsystem
  Sum : Sum  Inputs=++|
  rate_dot_cmd_B : Outport
  wires:
  INS_Out/1 -> Error/2(INS_Out)
  Error/1(rate_err_radPs) -> PID_Controller/1(rate_err_radPs)
  rate_cmd_radPs/1 -> Feedforward_Controller/1(rate_cmd_radPs), Error/1(rate_cmd_radPs)
  reset/1 -> PID_Controller/2(reset)
  PID_Controller/1(rate_dot_cmd_B) -> Sum/2
  Sum/1 -> rate_dot_cmd_B/1
  Feedforward_Controller/1(rate_dot_cmd_B) -> Sum/1

== system Controller/Controller/Horizontal_Control/Attitude_Controller/Inner_Loop/Signal_Convert ==
  FMS_Out : Inport
  euler_rate_cmd : Inport  Port=2
  INS_Out : Inport  Port=3
  Bus Selector2 : BusSelector  OutputSignals=psi_rate_cmd
  Bus Selector3 : BusSelector  OutputSignals=phi,theta
  Euler To Angle Rate : FMT_Model_Lib/Math/Euler To Angle Rate
      settings: SourceProductName=FMT Toolbox
  Mux1 : Mux  Inputs=2
  Mux2 : Mux  Inputs=2
  Saturation : Saturate  UpperLimit=CONTROL_PARAM.MC_RATE_Z_LIM  LowerLimit=-CONTROL_PARAM.MC_RATE_Z_LIM
  Saturation1 : Saturate  UpperLimit=CONTROL_PARAM.MC_RATE_XY_LIM  LowerLimit=-CONTROL_PARAM.MC_RATE_XY_LIM
  rate_cmd_radPs : Outport
  wires:
  Bus Selector3/1 -> Mux2/1  "<phi>"
  Mux2/1 -> Euler To Angle Rate/1
  Bus Selector3/2 -> Mux2/2  "<theta>"
  euler_rate_cmd/1 -> Saturation1/1
  Bus Selector2/1 -> Saturation/1  "<psi_rate_cmd>"
  Mux1/1 -> Euler To Angle Rate/2  "euler_rate"
  FMS_Out/1 -> Bus Selector2/1
  INS_Out/1 -> Bus Selector3/1
  Euler To Angle Rate/1 -> rate_cmd_radPs/1  "ang_rate"
  Saturation/1 -> Mux1/2
  Saturation1/1 -> Mux1/1

== system Controller/Controller/Horizontal_Control/Attitude_Controller/Inner_Loop/Signal_Select ==
  note: mode:
      | 0: Unknown
      | 1: Mission
      | 2: Stablize
      | 3: Altitude Hold
      | 4: Attitude Mode
      | 5: Acro Mode
  FMS_Out : Inport
  rate_cmd_radPs : Inport  Port=2
  Bus Selector : BusSelector  OutputSignals=ctrl_mode
  Bus Selector1 : BusSelector  OutputSignals=p_cmd,q_cmd,r_cmd
  Compare To Constant : simulink/Logic and Bit Operations/Compare To Constant  relop===  const=uint8(ControlMode.Acro)  OutDataTypeStr=boolean
  Compare To Constant1 : simulink/Logic and Bit Operations/Compare To Constant  relop===  const=uint8(ControlMode.Offboard)  OutDataTypeStr=boolean
  Mux : Mux  Inputs=3
  Offboard_Signal_Select : Subsystem
  Switch : Switch  Criteria=u2 > Threshold
  Switch1 : Switch  Criteria=u2 > Threshold
  out : Outport
  wires:
  FMS_Out/1 -> Bus Selector/1, Offboard_Signal_Select/1(FMS_Out), Bus Selector1/1
  Switch/1 -> out/1
  Bus Selector/1 -> Compare To Constant1/1, Compare To Constant/1  "<ctrl_mode>"
  Compare To Constant/1 -> Switch/2
  Bus Selector1/1 -> Mux/1  "<p_cmd>"
  Bus Selector1/2 -> Mux/2  "<q_cmd>"
  Bus Selector1/3 -> Mux/3  "<r_cmd>"
  Mux/1 -> Switch/1
  rate_cmd_radPs/1 -> Switch1/3, Offboard_Signal_Select/2(rate_cmd_in)
  Switch1/1 -> Switch/3
  Offboard_Signal_Select/1(rate_cmd_radPs) -> Switch1/1
  Compare To Constant1/1 -> Switch1/2

== system Controller/Controller/Horizontal_Control/Attitude_Controller/Outter_Loop/Attitude_Controller ==
  att_cmd_rad : Inport
  INS_Out : Inport  Port=2
  Error : Subsystem
  Sqrt_Root_Controller : Subsystem
  euler_rate_cmd_radPs : Outport
  wires:
  INS_Out/1 -> Error/2(INS_Out)
  Sqrt_Root_Controller/1(euler_rate_cmd_radPs) -> euler_rate_cmd_radPs/1
  att_cmd_rad/1 -> Error/1(att_cmd)
  Error/1(euler_err_rad) -> Sqrt_Root_Controller/1(euler_err_rad)

== system Controller/Controller/Horizontal_Control/Attitude_Controller/Outter_Loop/Signal_Select ==
  note: mode:
      | 0: Unknown
      | 1: Mission
      | 2: Position
      | 3: Altitude Hold
      | 4: Manual Mode
      | 5: Acro Mode
      | 6: Offboard
  att_cmd_rad : Inport
  FMS_Out : Inport  Port=2
  Bus Selector : BusSelector  OutputSignals=ctrl_mode
  Bus Selector1 : BusSelector  OutputSignals=phi_cmd,theta_cmd
  Compare To Constant : simulink/Logic and Bit Operations/Compare To Constant  relop===  const=uint8([ControlMode.Stabilize, ControlMode.ALTCTL])  OutDataTypeStr=boolean
  Compare To Constant1 : simulink/Logic and Bit Operations/Compare To Constant  relop===  const=uint8(ControlMode.Offboard)  OutDataTypeStr=boolean
  Logical Operator : Logic  Operator=OR  Inputs=1  AllPortsSameDT=off  OutDataTypeStr=boolean
  Mux : Mux  Inputs=2
  Offboard_Signal_Select : Subsystem
  Switch : Switch  Criteria=u2 > Threshold
  Switch1 : Switch  Criteria=u2 > Threshold
  out : Outport
  wires:
  Compare To Constant/1 -> Logical Operator/1
  Bus Selector1/2 -> Mux/2  "<theta_cmd>"
  Bus Selector1/1 -> Mux/1  "<phi_cmd>"
  Bus Selector/1 -> Compare To Constant1/1, Compare To Constant/1  "<ctrl_mode>"
  FMS_Out/1 -> Bus Selector/1, Bus Selector1/1, Offboard_Signal_Select/1(FMS_Out)
  Mux/1 -> Switch/1
  Switch/1 -> out/1
  Logical Operator/1 -> Switch/2
  Switch1/1 -> Switch/3
  Compare To Constant1/1 -> Switch1/2
  Offboard_Signal_Select/1(att_cmd_rad) -> Switch1/1
  att_cmd_rad/1 -> Offboard_Signal_Select/2(att_cmd_in), Switch1/3

== system Controller/Controller/Horizontal_Control/Velocity_Controller/Error/Bus_Select ==
  INS_Out : Inport
  Bus Selector1 : BusSelector  OutputSignals=vn,ve
  Bus Selector2 : BusSelector  OutputSignals=psi
  Constant : Constant  Value=0  OutDataTypeStr=single
  Multiply : Product  Multiplication=Matrix(*)
  Mux2 : Mux  Inputs=3
  Psi To DCM : FMT_Model_Lib/Transformation/Psi To DCM
      settings: SourceProductName=FMT Toolbox
  Selector : Selector  InputPortWidth=3  IndexOptions=Index vector (dialog)  Indices=[1 2]  OutputSizes=1
  uv_est_C_mPs : Outport
  wires:
  Psi To DCM/1 -> Multiply/1
  Bus Selector2/1 -> Psi To DCM/1  "<psi>"
  Bus Selector1/2 -> Mux2/2  "<ve>"
  Bus Selector1/1 -> Mux2/1  "<vn>"
  INS_Out/1 -> Bus Selector2/1, Bus Selector1/1
  Mux2/1 -> Multiply/2
  Selector/1 -> uv_est_C_mPs/1
  Constant/1 -> Mux2/3  "<velD>"
  Multiply/1 -> Selector/1

== system Controller/Controller/Horizontal_Control/Velocity_Controller/Error/TD ==
  v : Inport
  v0 : Inport  Port=2
  Integrator : DiscreteIntegrator  SampleTime=-1  ICPrevOutput=DiscIntNeverNeededParam  ICPrevScaledInput=DiscIntNeverNeededParam
  Integrator1 : DiscreteIntegrator  InitialConditionSource=external  SampleTime=-1  ICPrevOutput=DiscIntNeverNeededParam  ICPrevScaledInput=DiscIntNeverNeededParam
  Subtract : Sum  Inputs=+-
  "fhan " : Subsystem  mask{r0=6*9.806, h0=0.05}
      mask DialogControl ParameterGroupVar Prompt: fhan(v1,v2,r0,h0)
  v1 : Outport
  wires:
  Integrator1/1 -> Subtract/1, v1/1
  v/1 -> Subtract/2
  Integrator/1 -> "fhan "/2(v2), Integrator1/1  "v2"
  Subtract/1 -> "fhan "/1(v1)
  "fhan "/1(fhan) -> Integrator/1
  v0/1 -> Integrator1/2

== system Controller/Controller/Horizontal_Control/Velocity_Controller/PID_Controller/D_Control ==
  err : Inport
  reset : Inport  Port=2
  DT Filter : FMT_Model_Lib/Filter/DT Filter  fc=10
      settings: SourceProductName=FMT Toolbox
  Multiply : Product  OutDataTypeStr=Inherit: Same as first input
  Saturation : Saturate  UpperLimit=max_d  LowerLimit=min_d
  kd : Constant  Value=kd  OutDataTypeStr=single
  d_out : Outport
  wires:
  err/1 -> DT Filter/1
  kd/1 -> Multiply/1
  Multiply/1 -> Saturation/1
  Saturation/1 -> d_out/1
  reset/1 -> DT Filter/2
  DT Filter/1 -> Multiply/2

== system Controller/Controller/Horizontal_Control/Velocity_Controller/PID_Controller/I_Control ==
  err : Inport
  reset : Inport  Port=2
  Constant : Constant  Value=0  OutDataTypeStr=single
  Discrete-Time Integrator : DiscreteIntegrator  ExternalReset=level  InitialConditionSource=external  SampleTime=-1  LimitOutput=on  UpperSaturationLimit=max_i  LowerSaturationLimit=min_i  ICPrevOutput=DiscIntNeverNeededParam  ICPrevScaledInput=DiscIntNeverNeededParam
  Multiply : Product  OutDataTypeStr=Inherit: Same as first input
  ki : Constant  Value=ki  OutDataTypeStr=single
  i_out : Outport
  wires:
  err/1 -> Multiply/2
  Multiply/1 -> Discrete-Time Integrator/1
  reset/1 -> Discrete-Time Integrator/2
  Constant/1 -> Discrete-Time Integrator/3
  Discrete-Time Integrator/1 -> i_out/1
  ki/1 -> Multiply/1

== system Controller/Controller/Horizontal_Control/Velocity_Controller/PID_Controller/P_Control ==
  err : Inport
  Multiply : Product  OutDataTypeStr=Inherit: Same as first input
  kp : Constant  Value=kp  OutDataTypeStr=single
  p_out : Outport
  wires:
  err/1 -> Multiply/2
  kp/1 -> Multiply/1
  Multiply/1 -> p_out/1

== system Controller/Controller/Horizontal_Control/Velocity_Controller/Signal_Select/Offboard_Signal_Select ==
  FMS_Out : Inport
  acc_cmd_in : Inport  Port=2
  Bus Selector1 : BusSelector  OutputSignals=cmd_mask
  Bus Selector2 : BusSelector  OutputSignals=ax_cmd,ay_cmd
  Compare To Zero : simulink/Logic and Bit Operations/Compare To Zero  relop=>  OutDataTypeStr=boolean
  Compare To Zero2 : simulink/Logic and Bit Operations/Compare To Zero  relop=>  OutDataTypeStr=boolean
  Multiply2 : Product
  Multiply3 : Product
  Mux : Mux  Inputs=2
  Mux1 : Mux  Inputs=2
  Mux2 : Mux  Inputs=2
  Sum1 : Sum  Inputs=|++
  cmd_ax valid : simulink/Logic and Bit Operations/Bitwise Operator  logicop=AND  UseBitMask=on  BitMask=bin2dec('1000000000')  BitMaskRealWorld=Stored Integer
  cmd_ay valid : simulink/Logic and Bit Operations/Bitwise Operator  logicop=AND  UseBitMask=on  BitMask=bin2dec('10000000000')  BitMaskRealWorld=Stored Integer
  cmd_u valid : simulink/Logic and Bit Operations/Bitwise Operator  logicop=AND  UseBitMask=on  BitMask=bin2dec('1000000')  BitMaskRealWorld=Stored Integer
  cmd_v valid : simulink/Logic and Bit Operations/Bitwise Operator  logicop=AND  UseBitMask=on  BitMask=bin2dec('10000000')  BitMaskRealWorld=Stored Integer
  acc_cmd : Outport
  wires:
  Multiply2/1 -> Sum1/2
  FMS_Out/1 -> Bus Selector2/1, Bus Selector1/1
  Bus Selector1/1 -> cmd_v valid/1, cmd_u valid/1, cmd_ay valid/1, cmd_ax valid/1  "<cmd_mask>"
  Multiply3/1 -> Sum1/1
  cmd_u valid/1 -> Mux1/1
  cmd_v valid/1 -> Mux1/2
  Mux1/1 -> Compare To Zero/1
  acc_cmd_in/1 -> Multiply2/2
  Compare To Zero/1 -> Multiply2/1
  Bus Selector2/1 -> Mux/1  "<ax_cmd>"
  cmd_ax valid/1 -> Mux2/1
  cmd_ay valid/1 -> Mux2/2
  Mux2/1 -> Compare To Zero2/1
  Compare To Zero2/1 -> Multiply3/2
  Bus Selector2/2 -> Mux/2  "<ay_cmd>"
  Mux/1 -> Multiply3/1
  Sum1/1 -> acc_cmd/1

== system Controller/Controller/Vertical_Control/Veloxity_Z_Controller/Error/TD ==
  v : Inport
  v0 : Inport  Port=2
  Integrator : DiscreteIntegrator  SampleTime=-1  ICPrevOutput=DiscIntNeverNeededParam  ICPrevScaledInput=DiscIntNeverNeededParam
  Integrator1 : DiscreteIntegrator  InitialConditionSource=external  SampleTime=-1  ICPrevOutput=DiscIntNeverNeededParam  ICPrevScaledInput=DiscIntNeverNeededParam
  Subtract : Sum  Inputs=+-
  "fhan " : Subsystem  mask{r0=8*9.806, h0=0.05}
      mask DialogControl ParameterGroupVar Prompt: fhan(v1,v2,r0,h0)
  v1 : Outport
  wires:
  Integrator1/1 -> Subtract/1, v1/1
  v/1 -> Subtract/2
  Integrator/1 -> "fhan "/2(v2), Integrator1/1  "v2"
  Subtract/1 -> "fhan "/1(v1)
  "fhan "/1(fhan) -> Integrator/1
  v0/1 -> Integrator1/2

== system Controller/Controller/Vertical_Control/Veloxity_Z_Controller/PID_Controller/D_Control ==
  err : Inport
  reset : Inport  Port=2
  DT Filter : FMT_Model_Lib/Filter/DT Filter  fc=10
      settings: SourceProductName=FMT Toolbox
  Multiply : Product  OutDataTypeStr=Inherit: Same as first input
  Saturation : Saturate  UpperLimit=max_d  LowerLimit=min_d
  kd : Constant  Value=kd  OutDataTypeStr=single
  d_out : Outport
  wires:
  err/1 -> DT Filter/1
  kd/1 -> Multiply/1
  Multiply/1 -> Saturation/1
  Saturation/1 -> d_out/1
  reset/1 -> DT Filter/2
  DT Filter/1 -> Multiply/2

== system Controller/Controller/Vertical_Control/Veloxity_Z_Controller/PID_Controller/I_Control ==
  err : Inport
  slow_start : Inport  Port=2
  reset : Inport  Port=3
  Constant : Constant  Value=min_i  OutDataTypeStr=single
  Constant1 : Constant  Value=0  OutDataTypeStr=single
  Discrete-Time Integrator : DiscreteIntegrator  ExternalReset=level  InitialConditionSource=external  SampleTime=-1  LimitOutput=on  UpperSaturationLimit=max_i  LowerSaturationLimit=min_i  ICPrevOutput=DiscIntNeverNeededParam  ICPrevScaledInput=DiscIntNeverNeededParam
  Multiply : Product  OutDataTypeStr=Inherit: Same as first input
  Switch : Switch  Criteria=u2 > Threshold
  ki : Constant  Value=ki  OutDataTypeStr=single
  i_out : Outport
  wires:
  err/1 -> Multiply/2
  Multiply/1 -> Discrete-Time Integrator/1
  reset/1 -> Discrete-Time Integrator/2
  Switch/1 -> Discrete-Time Integrator/3
  Discrete-Time Integrator/1 -> i_out/1
  ki/1 -> Multiply/1
  slow_start/1 -> Switch/2
  Constant/1 -> Switch/1
  Constant1/1 -> Switch/3

== system Controller/Controller/Vertical_Control/Veloxity_Z_Controller/PID_Controller/P_Control ==
  err : Inport
  Multiply : Product  OutDataTypeStr=Inherit: Same as first input
  kp : Constant  Value=kp  OutDataTypeStr=single
  p_out : Outport
  wires:
  err/1 -> Multiply/2
  kp/1 -> Multiply/1
  Multiply/1 -> p_out/1

== system Controller/Controller/Horizontal_Control/Attitude_Controller/Inner_Loop/Rate_Controller/Error ==
  rate_cmd_radPs : Inport
  INS_Out : Inport  Port=2
  Bus_Select : Subsystem
  First Order LPF : FMT_Model_Lib/Filter/First Order LPF  fc=30
      settings: SourceProductName=FMT Toolbox
  Sum : Sum  Inputs=|+-
  rate_err_radPs : Outport
  wires:
  Sum/1 -> First Order LPF/1  "rate_error_B_radPs"
  rate_cmd_radPs/1 -> Sum/1  "rate_cmd_B_radPs"
  INS_Out/1 -> Bus_Select/1(INS_Out)
  Bus_Select/1(rate_est_radPs) -> Sum/2  "rate_est_B_radPs"
  First Order LPF/1 -> rate_err_radPs/1

== system Controller/Controller/Horizontal_Control/Attitude_Controller/Inner_Loop/Rate_Controller/Feedforward_Controller ==
  rate_cmd_radPs : Inport
  DeadZone : Subsystem  mask{th=0.1}
      mask prompts: th "Threshold"
      mask Display: disp('Dead Zone')
  Demux : Demux  Outputs=3
  Gain : Gain  Gain=CONTROL_PARAM.MC_ROLLRATE_FF
  Gain1 : Gain  Gain=CONTROL_PARAM.MC_PITCHRATE_FF
  Gain2 : Gain  Gain=CONTROL_PARAM.MC_YAWRATE_FF
  Mux : Mux  Inputs=3
  rate_dot_cmd_B : Outport
  wires:
  rate_cmd_radPs/1 -> DeadZone/1(u)
  Demux/2 -> Gain1/1
  Demux/1 -> Gain/1
  Gain1/1 -> Mux/2
  DeadZone/1(y) -> Demux/1
  Mux/1 -> rate_dot_cmd_B/1  "rate_dot_ff_cmd"
  Gain/1 -> Mux/1
  Demux/3 -> Gain2/1
  Gain2/1 -> Mux/3
